simulink model "IEEE33_TR_TEMPORAL_RECOGNIZABILITY_MASTER"  (R2026b)
settings: Solver=ode23t  StopTime=0.2  MaxStep=1e-5
undefined symbols (not defined in the file): Three_PhaseBreaker_class, Three_PhaseSeriesRLCLoad_class, Three_PhaseSource_class, Three_PhaseV_IMeasuremen_class
libraries: ee_lib x146, nesl_utility x106, fl_lib x33, eeRmsMeasurement x2
(part 1 of 7)
settings Model: Creator=JY Wong  LastModifiedBy=sola
settings DataIOCC: ReturnWorkspaceOutputs=off
settings DebuggingCC: ArithmeticOperatorsInVariantConditions=warning  PregeneratedLibrarySubsystemCodeDiagnostic=none  SaveWithParameterizedLinksMsg=none
settings SFSimCC: CustomCodeUndefinedFunction=UseInterfaceOnly  SimUseLocalCustomCode=off
settings RTWCC: RTWUseLocalCustomCode=off
settings SimscapeCC: SimscapeNominalValues="[{\"value\":\"1\",\"unit\":\"A\"},{\"value\":\"1\",\"unit\":\"bar\"},{\"value\":\"1\",\"unit\":\"cm^2\"},{\"value\":\"1\",\"unit\":\"cm^3/s\"},{\"value\":\"1\",\"unit\":\"kJ/kg\"},{\"value\":\"1\",\"unit\":\"kW\"},{\"value\":\"1\",\"unit\":\"l\"},{\"value\":\"1\",\"unit\":\"N\"},{\"value\":\"1\",\"unit\":\"N*m\"},{\"value\":\"1\",\"unit\":\"V\"},{\"value\":\"0.001\",\"unit\":\"Wb\"}]"  SimscapeUseEnergyAccounting=off

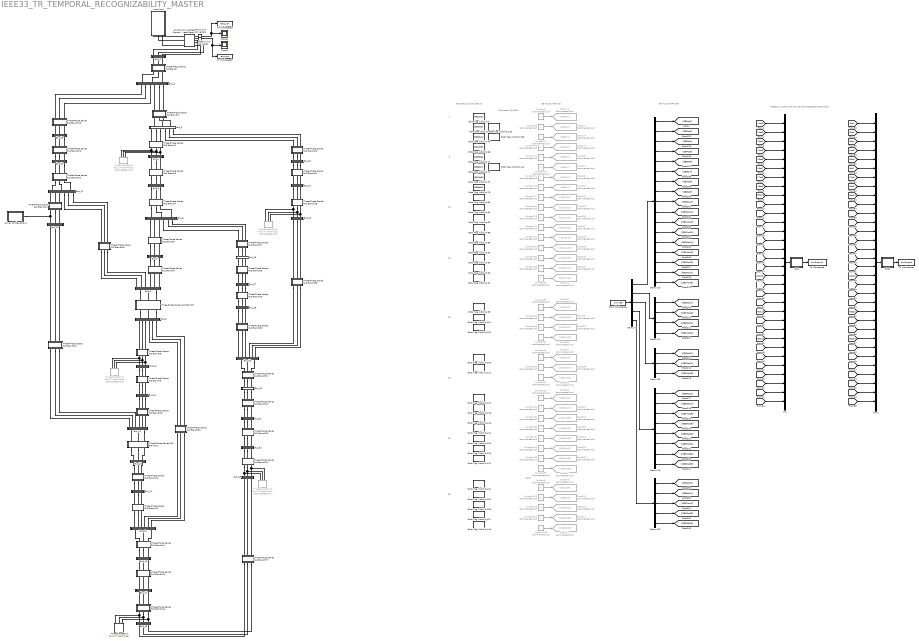
== system IEEE33_TR_TEMPORAL_RECOGNIZABILITY_MASTER ==
  note: NoPs
  note: 33 buses + 5 NOPs
  note: Goto Tag Visibility Blocks
  note: 1
  note: 5
  note: 10
  note: 15
  note: 20
  note: 25
  note: 30
  note: CB Inputs (Manual)
  note: CB Inputs (MATLAB)
  note: Voltage & Current Monitoring at the Respective Branches
  note: 35
  Bus_1 : Subsystem
  Bus_10 : Subsystem
  Bus_11 : Subsystem
  Bus_12 : Subsystem
  Bus_13 : Subsystem
  Bus_14 : Subsystem
  Bus_15 : Subsystem
  Bus_16 : Subsystem
  Bus_17 : Subsystem
  Bus_18 : Subsystem
  Bus_19 : Subsystem
  Bus_2 : Subsystem
  Bus_20 : Subsystem
  Bus_21 : Subsystem
  Bus_22 : Subsystem
  Bus_23 : Subsystem
  Bus_24 : Subsystem
  Bus_25 : Subsystem
  Bus_26 : Subsystem
  Bus_27 : Subsystem
  Bus_28 : Subsystem
  Bus_29 : Subsystem
  Bus_3 : Subsystem
  Bus_30 : Subsystem
  Bus_31 : Subsystem
  Bus_32 : Subsystem
  Bus_33 : Subsystem
  Bus_4 : Subsystem
  Bus_5 : Subsystem
  Bus_6 : Subsystem
  Bus_7 : Subsystem
  Bus_8 : Subsystem
  Bus_9 : Subsystem
  Constant{7..8,71..100} (32 alike) : Constant  Commented=on
  Constant{3..4,133..135} (5 alike) : Constant  Commented=on  Value=0
  Current and Voltage Sensor (Three-Phase) : ee_lib/Sensors & Transducers/Current and Voltage Sensor (Three-Phase)  port_option=ee.enum.threePhasePort.expanded  vMeasurementType=ee.enum.vmeasurement.lg  outputUnit=ee.enum.unit.si  SRated=100e6 A*V  VRated=24e3 V  I_specify=off  I_priority=None  I=[0, 0, 0] A  I_nominal_specify=off  I_nominal_value=1  I_nominal_unit=A  V_specify=off  V_priority=None  V=[0, 0, 0] V  V_nominal_specify=off  V_nominal_value=1  V_nominal_unit=V
  Demux1 : Demux  Outputs=[17,4,3,8,5]
  Demux13 : Demux  Outputs=17
  Demux14 : Demux
  Demux15 : Demux  Outputs=3
  Demux16 : Demux  Outputs=8
  Demux20 : Demux  Outputs=5
  From Workspace1 : FromWorkspace  VariableName=siminCB
  Goto Tag Visibility : GotoTagVisibility  GotoTag=CB2to3
  Goto Tag Visibility102 : GotoTagVisibility  GotoTag=CB21to22
  Goto Tag Visibility104 : GotoTagVisibility  GotoTag=CB20to21
  Goto Tag Visibility106 : GotoTagVisibility  GotoTag=CB23to24
  Goto Tag Visibility110 : GotoTagVisibility  GotoTag=CB26to27
  Goto Tag Visibility112 : GotoTagVisibility  GotoTag=CB24to25
  Goto Tag Visibility114 : GotoTagVisibility  GotoTag=CB6to26
  Goto Tag Visibility116 : GotoTagVisibility  GotoTag=CB28to29
  Goto Tag Visibility118 : GotoTagVisibility  GotoTag=CB27to28
  Goto Tag Visibility120 : GotoTagVisibility  GotoTag=CB30to31
  Goto Tag Visibility122 : GotoTagVisibility  GotoTag=CB29to30
  Goto Tag Visibility124 : GotoTagVisibility  GotoTag=CB32to33
  Goto Tag Visibility126 : GotoTagVisibility  GotoTag=CB31to32
  Goto Tag Visibility129 : GotoTagVisibility  GotoTag=CB2to19
  Goto Tag Visibility130 : GotoTagVisibility  GotoTag=CB3to23
  Goto Tag Visibility132 : GotoTagVisibility  GotoTag=CB9to15
  Goto Tag Visibility134 : GotoTagVisibility  GotoTag=CB21to8
  Goto Tag Visibility136 : GotoTagVisibility  GotoTag=CB22to12
  Goto Tag Visibility137 : GotoTagVisibility  GotoTag=CB18to33
  Goto Tag Visibility140 : GotoTagVisibility  GotoTag=CB25to29
  Goto Tag Visibility4 : GotoTagVisibility  GotoTag=CB1to2
  Goto Tag Visibility68 : GotoTagVisibility  GotoTag=CB4to5
  Goto Tag Visibility70 : GotoTagVisibility  GotoTag=CB3to4
  Goto Tag Visibility72 : GotoTagVisibility  GotoTag=CB6to7
  Goto Tag Visibility74 : GotoTagVisibility  GotoTag=CB5to6
  Goto Tag Visibility76 : GotoTagVisibility  GotoTag=CB8to9
  Goto Tag Visibility78 : GotoTagVisibility  GotoTag=CB7to8
  Goto Tag Visibility80 : GotoTagVisibility  GotoTag=CB9to10
  Goto Tag Visibility82 : GotoTagVisibility  GotoTag=CB11to12
  Goto Tag Visibility84 : GotoTagVisibility  GotoTag=CB10to11
  Goto Tag Visibility86 : GotoTagVisibility  GotoTag=CB13to14
  Goto Tag Visibility88 : GotoTagVisibility  GotoTag=CB12to13
  Goto Tag Visibility90 : GotoTagVisibility  GotoTag=CB15to16
  Goto Tag Visibility92 : GotoTagVisibility  GotoTag=CB14to15
  Goto Tag Visibility94 : GotoTagVisibility  GotoTag=CB17to18
  Goto Tag Visibility96 : GotoTagVisibility  GotoTag=CB16to17
  Goto Tag Visibility98 : GotoTagVisibility  GotoTag=CB19to20
  Goto276 : Goto  Commented=on  GotoTag=CB1to2  TagVisibility=scoped
  Goto277 : Goto  Commented=on  GotoTag=CB2to3  TagVisibility=scoped
  Goto278 : Goto  Commented=on  GotoTag=CB3to4  TagVisibility=scoped
  Goto279 : Goto  Commented=on  GotoTag=CB4to5  TagVisibility=scoped
  Goto280 : Goto  Commented=on  GotoTag=CB5to6  TagVisibility=scoped
  Goto281 : Goto  Commented=on  GotoTag=CB6to7  TagVisibility=scoped
  Goto282 : Goto  Commented=on  GotoTag=CB7to8  TagVisibility=scoped
  Goto283 : Goto  Commented=on  GotoTag=CB8to9  TagVisibility=scoped
  Goto284 : Goto  Commented=on  GotoTag=CB9to10  TagVisibility=scoped
  Goto285 : Goto  Commented=on  GotoTag=CB10to11  TagVisibility=scoped
  Goto286 : Goto  Commented=on  GotoTag=CB11to12  TagVisibility=scoped
  Goto287 : Goto  Commented=on  GotoTag=CB12to13  TagVisibility=scoped
  Goto288 : Goto  Commented=on  GotoTag=CB13to14  TagVisibility=scoped
  Goto289 : Goto  Commented=on  GotoTag=CB14to15  TagVisibility=scoped
  Goto290 : Goto  Commented=on  GotoTag=CB15to16  TagVisibility=scoped
  Goto291 : Goto  Commented=on  GotoTag=CB16to17  TagVisibility=scoped
  Goto292 : Goto  Commented=on  GotoTag=CB2to19  TagVisibility=scoped
  Goto293 : Goto  Commented=on  GotoTag=CB19to20  TagVisibility=scoped
  Goto294 : Goto  Commented=on  GotoTag=CB20to21  TagVisibility=scoped
  Goto295 : Goto  Commented=on  GotoTag=CB21to22  TagVisibility=scoped
  Goto296 : Goto  Commented=on  GotoTag=CB17to18  TagVisibility=scoped
  Goto297 : Goto  Commented=on  GotoTag=CB3to23  TagVisibility=scoped
  Goto298 : Goto  Commented=on  GotoTag=CB23to24  TagVisibility=scoped
  Goto299 : Goto  Commented=on  GotoTag=CB24to25  TagVisibility=scoped
  Goto300 : Goto  Commented=on  GotoTag=CB6to26  TagVisibility=scoped
  Goto301 : Goto  Commented=on  GotoTag=CB26to27  TagVisibility=scoped
  Goto302 : Goto  Commented=on  GotoTag=CB27to28  TagVisibility=scoped
  Goto303 : Goto  Commented=on  GotoTag=CB28to29  TagVisibility=scoped
  Goto304 : Goto  Commented=on  GotoTag=CB29to30  TagVisibility=scoped
  Goto305 : Goto  Commented=on  GotoTag=CB30to31  TagVisibility=scoped
  Goto306 : Goto  Commented=on  GotoTag=CB31to32  TagVisibility=scoped
  Goto307 : Goto  Commented=on  GotoTag=CB32to33  TagVisibility=scoped
  Goto308 : Goto  Commented=on  GotoTag=CB21to8  TagVisibility=scoped
  Goto309 : Goto  Commented=on  GotoTag=CB9to15  TagVisibility=scoped
  Goto310 : Goto  Commented=on  GotoTag=CB22to12  TagVisibility=scoped
  Goto311 : Goto  Commented=on  GotoTag=CB18to33  TagVisibility=scoped
  Goto312 : Goto  Commented=on  GotoTag=CB25to29  TagVisibility=scoped
  Incoming1 : Subsystem
  Mux : Mux  Inputs=32
  Mux1 : Mux  Inputs=32
  PS-Simulink Converter : nesl_utility/PS-Simulink Converter  PhysicalDomain=network_engine_domain  SubClassName=ps_output  LeftPortType=input  RightPortType=output  PseudoPeriodic=off  Frequencies=[]  VectorFormat=inherit  Unit=inherit  AffineConversion=off
  PS-Simulink Converter1 : nesl_utility/PS-Simulink Converter  PhysicalDomain=network_engine_domain  SubClassName=ps_output  LeftPortType=input  RightPortType=output  PseudoPeriodic=off  Frequencies=[]  VectorFormat=inherit  Unit=inherit  AffineConversion=off
  RMS : Subsystem
      settings: OpenFcn=elec.conv.unmask(gcb);
  RMS1 : Subsystem
      settings: OpenFcn=elec.conv.unmask(gcb);
  Scope : Scope
      settings: ActiveDisplayYMinimum=-377.76200799670079  ActiveDisplayYMaximum=376.93956006483484
  Scope1 : Scope
      settings: ActiveDisplayYMinimum=-12921.058393181265  ActiveDisplayYMaximum=12921.058393181265
  Solver Configuration1 : Subsystem  Priority=1
  Three-Phase Series RLC Branch : Subsystem
      settings: AttributesFormatString=\n  OpenFcn=elec.conv.unmask(gcb);
  Three-Phase Series RLC Branch1 : Subsystem
      settings: AttributesFormatString=\n  OpenFcn=elec.conv.unmask(gcb);
  Three-Phase Series RLC Branch10 : Subsystem
      settings: AttributesFormatString=\n  OpenFcn=elec.conv.unmask(gcb);
  Three-Phase Series RLC Branch11 : Subsystem
      settings: AttributesFormatString=\n  OpenFcn=elec.conv.unmask(gcb);
  Three-Phase Series RLC Branch12 : Subsystem
      settings: AttributesFormatString=\n  OpenFcn=elec.conv.unmask(gcb);
  Three-Phase Series RLC Branch13 : Subsystem
      settings: AttributesFormatString=\n  OpenFcn=elec.conv.unmask(gcb);
  Three-Phase Series RLC Branch14 : Subsystem
      settings: AttributesFormatString=\n  OpenFcn=elec.conv.unmask(gcb);
  Three-Phase Series RLC Branch15 : Subsystem
      settings: AttributesFormatString=\n  OpenFcn=elec.conv.unmask(gcb);
  Three-Phase Series RLC Branch16 : Subsystem
      settings: AttributesFormatString=\n  OpenFcn=elec.conv.unmask(gcb);
  Three-Phase Series RLC Branch18 : Subsystem
      settings: AttributesFormatString=\n  OpenFcn=elec.conv.unmask(gcb);
  Three-Phase Series RLC Branch19 : Subsystem
      settings: AttributesFormatString=\n  OpenFcn=elec.conv.unmask(gcb);
  Three-Phase Series RLC Branch2 : Subsystem
      settings: AttributesFormatString=\n  OpenFcn=elec.conv.unmask(gcb);
  Three-Phase Series RLC Branch20 : Subsystem
      settings: AttributesFormatString=\n  OpenFcn=elec.conv.unmask(gcb);
  Three-Phase Series RLC Branch21 : Subsystem
      settings: AttributesFormatString=\n  OpenFcn=elec.conv.unmask(gcb);
  Three-Phase Series RLC Branch22 : Subsystem
      settings: AttributesFormatString=\n  OpenFcn=elec.conv.unmask(gcb);
  Three-Phase Series RLC Branch23 : Subsystem
      settings: AttributesFormatString=\n  OpenFcn=elec.conv.unmask(gcb);
  Three-Phase Series RLC Branch24 : Subsystem
      settings: AttributesFormatString=\n  OpenFcn=elec.conv.unmask(gcb);
  Three-Phase Series RLC Branch25 : Subsystem
      settings: AttributesFormatString=\n  OpenFcn=elec.conv.unmask(gcb);
  Three-Phase Series RLC Branch27 : Subsystem
      settings: AttributesFormatString=\n  OpenFcn=elec.conv.unmask(gcb);
  Three-Phase Series RLC Branch28 : Subsystem
      settings: AttributesFormatString=\n  OpenFcn=elec.conv.unmask(gcb);
  Three-Phase Series RLC Branch29 : Subsystem
      settings: AttributesFormatString=\n  OpenFcn=elec.conv.unmask(gcb);
  Three-Phase Series RLC Branch3 : Subsystem
      settings: AttributesFormatString=\n  OpenFcn=elec.conv.unmask(gcb);
  Three-Phase Series RLC Branch30 : Subsystem
      settings: AttributesFormatString=\n  OpenFcn=elec.conv.unmask(gcb);
  Three-Phase Series RLC Branch31 : Subsystem
      settings: AttributesFormatString=\n  OpenFcn=elec.conv.unmask(gcb);
  Three-Phase Series RLC Branch32 : Subsystem
      settings: AttributesFormatString=\n  OpenFcn=elec.conv.unmask(gcb);
  Three-Phase Series RLC Branch33 : Subsystem
      settings: AttributesFormatString=\n  OpenFcn=elec.conv.unmask(gcb);
  Three-Phase Series RLC Branch34 : Subsystem
      settings: AttributesFormatString=\n  OpenFcn=elec.conv.unmask(gcb);
  Three-Phase Series RLC Branch35 : Subsystem
      settings: AttributesFormatString=\n  OpenFcn=elec.conv.unmask(gcb);
  Three-Phase Series RLC Branch36 : Subsystem
      settings: AttributesFormatString=\n  OpenFcn=elec.conv.unmask(gcb);
  Three-Phase Series RLC Branch37 : Subsystem
      settings: AttributesFormatString=\n  OpenFcn=elec.conv.unmask(gcb);
  Three-Phase Series RLC Branch38 : Subsystem
      settings: AttributesFormatString=\n  OpenFcn=elec.conv.unmask(gcb);
  Three-Phase Series RLC Branch4 : Subsystem
      settings: AttributesFormatString=\n  OpenFcn=elec.conv.unmask(gcb);
  Three-Phase Series RLC Branch5 : Subsystem
      settings: AttributesFormatString=\n  OpenFcn=elec.conv.unmask(gcb);
  Three-Phase Series RLC Branch6 : Subsystem
      settings: AttributesFormatString=\n  OpenFcn=elec.conv.unmask(gcb);
  Three-Phase Series RLC Branch7 : Subsystem
      settings: AttributesFormatString=\n  OpenFcn=elec.conv.unmask(gcb);
  Three-Phase Series RLC Branch8 : Subsystem
      settings: AttributesFormatString=\n  OpenFcn=elec.conv.unmask(gcb);
  Three-Phase Series RLC Branch9 : Subsystem
      settings: AttributesFormatString=\n  OpenFcn=elec.conv.unmask(gcb);
  ThreePhaseFault : ee_lib/Utilities/Fault (Three-Phase)  port_option=ee.enum.threePhasePort.expanded  fault_type_option=ee.enum.fault_type_option.none  R_pn_fault=0.999 Ohm  R_ng_fault=0.001 Ohm  exposemeasurement=ee.enum.exposemeasurement.hidden  enable_external_fault=ee.enum.external_fault.hidden  fault_threshold=0.5  fault_condition=ee.enum.fault_condition.fgt  fault_resettable=ee.enum.enable.no  enable_temporal_fault=ee.enum.enable.yes  fault_start_time=0.1 s  fault_duration=inf s  G_parasitic=1e-4 1/Ohm  I_specify=off  I_priority=None  I=[0, 0, 0] A  I_nominal_specify=off  I_nominal_value=1  I_nominal_unit=A  i_ng_specify=off  i_ng_priority=None  i_ng=0 A  i_ng_nominal_specify=off  i_ng_nominal_value=1  i_ng_nominal_unit=A
  ThreePhaseFault{1..4} (4 alike) : ee_lib/Utilities/Fault (Three-Phase)  Commented=on  port_option=ee.enum.threePhasePort.expanded  fault_type_option=ee.enum.fault_type_option.none  R_pn_fault=0.999 Ohm  R_ng_fault=0.001 Ohm  exposemeasurement=ee.enum.exposemeasurement.hidden  enable_external_fault=ee.enum.external_fault.hidden  fault_threshold=0.5  fault_condition=ee.enum.fault_condition.fgt  fault_resettable=ee.enum.enable.no  enable_temporal_fault=ee.enum.enable.yes  fault_start_time=0.1 s  fault_duration=inf s  G_parasitic=1e-4 1/Ohm  I_specify=off  I_priority=None  I=[0, 0, 0] A  I_nominal_specify=off  I_nominal_value=1  I_nominal_unit=A  i_ng_specify=off  i_ng_priority=None  i_ng=0 A  i_ng_nominal_specify=off  i_ng_nominal_value=1  i_ng_nominal_unit=A
  To Workspace : ToWorkspace  VariableName=simOutputV  SaveFormat=Timeseries  SampleTime=-1
  To Workspace1 : ToWorkspace  VariableName=simOutputI  SaveFormat=Timeseries  SampleTime=-1
  To Workspace2 : ToWorkspace  VariableName=Iabc_raw  SaveFormat=Timeseries  SampleTime=-1
  To Workspace3 : ToWorkspace  VariableName=Vabc_raw  SaveFormat=Timeseries  SampleTime=-1
  tag scope: CB10to11=scoped, CB11to12=scoped, CB12to13=scoped, CB13to14=scoped, CB14to15=scoped, CB15to16=scoped, CB16to17=scoped, CB17to18=scoped, CB18to33=scoped, CB19to20=scoped, CB1to2=scoped, CB20to21=scoped, CB21to22=scoped, CB21to8=scoped, CB22to12=scoped, CB23to24=scoped, CB24to25=scoped, CB25to29=scoped, CB26to27=scoped, CB27to28=scoped, CB28to29=scoped, CB29to30=scoped, CB2to19=scoped, CB2to3=scoped, CB30to31=scoped, CB31to32=scoped, CB32to33=scoped, CB3to23=scoped, CB3to4=scoped, CB4to5=scoped, CB5to6=scoped, CB6to26=scoped, CB6to7=scoped, CB7to8=scoped, CB8to9=scoped, CB9to10=scoped, CB9to15=scoped
  wires:
  Constant7/1 -> Goto276/1
  Constant8/1 -> Goto277/1
  Constant71/1 -> Goto278/1
  Constant72/1 -> Goto279/1
  Constant73/1 -> Goto280/1
  Constant76/1 -> Goto281/1
  Constant75/1 -> Goto283/1
  Constant74/1 -> Goto282/1
  Constant77/1 -> Goto284/1
  Constant80/1 -> Goto285/1
  Constant79/1 -> Goto287/1
  Constant78/1 -> Goto286/1
  Constant81/1 -> Goto288/1
  Constant84/1 -> Goto289/1
  Constant83/1 -> Goto291/1
  Constant82/1 -> Goto290/1
  Constant85/1 -> Goto292/1
  Constant88/1 -> Goto293/1
  Constant87/1 -> Goto295/1
  Constant86/1 -> Goto294/1
  Constant91/1 -> Goto299/1
  Constant93/1 -> Goto298/1
  Constant90/1 -> Goto297/1
  Constant94/1 -> Goto302/1
  Constant95/1 -> Goto303/1
  Constant96/1 -> Goto301/1
  Constant92/1 -> Goto300/1
  Constant98/1 -> Goto306/1
  Constant99/1 -> Goto307/1
  Constant100/1 -> Goto305/1
  Constant97/1 -> Goto304/1
  Constant89/1 -> Goto296/1
  From Workspace1/1 -> Demux1/1
  Demux14/2 -> [CB19to20]
  Demux13/17 -> [CB17to18]
  Demux16/5 -> [CB29to30]
  Demux16/8 -> [CB32to33]
  Demux13/15 -> [CB15to16]
  Demux13/5 -> [CB5to6]
  Demux13/11 -> [CB11to12]
  Demux13/10 -> [CB10to11]
  Demux16/7 -> [CB31to32]
  Demux15/2 -> [CB23to24]
  Demux13/3 -> [CB3to4]
  Demux13/4 -> [CB4to5]
  Demux13/16 -> [CB16to17]
  Demux13/6 -> [CB6to7]
  Demux13/1 -> [CB1to2]
  Demux15/3 -> [CB24to25]
  Demux16/2 -> [CB26to27]
  Demux1/4 -> Demux16/1
  Demux13/13 -> [CB13to14]
  Demux14/1 -> [CB2to19]
  Demux13/8 -> [CB8to9]
  Demux1/1 -> Demux13/1
  Demux16/3 -> [CB27to28]
  Demux13/12 -> [CB12to13]
  Demux13/14 -> [CB14to15]
  Demux16/6 -> [CB30to31]
  Demux13/2 -> [CB2to3]
  Demux13/7 -> [CB7to8]
  Demux1/3 -> Demux15/1
  Demux14/3 -> [CB20to21]
  Demux16/1 -> [CB6to26]
  Demux1/2 -> Demux14/1
  Demux13/9 -> [CB9to10]
  Demux16/4 -> [CB28to29]
  Demux14/4 -> [CB21to22]
  Demux15/1 -> [CB3to23]
  Mux/1 -> RMS/1(In)
  RMS/1(RMS) -> To Workspace/1
  RMS1/1(RMS) -> To Workspace1/1
  Mux1/1 -> RMS1/1(In)
  [I4to5] -> Mux1/4
  [I24to25] -> Mux1/24
  [I6to26] -> Mux1/25
  [I26to27] -> Mux1/26
  [I5to6] -> Mux1/5
  [I7to8] -> Mux1/7
  [I6to7] -> Mux1/6
  [I8to9] -> Mux1/8
  [I9to10] -> Mux1/9
  [I10to11] -> Mux1/10
  [I17to18] -> Mux1/17
  [I2to19] -> Mux1/18
  [I27to28] -> Mux1/27
  [I28to29] -> Mux1/28
  [I3to4] -> Mux1/3
  [I29to30] -> Mux1/29
  [I31to32] -> Mux1/31
  [I30to31] -> Mux1/30
  [I32to33] -> Mux1/32
  [I19to20] -> Mux1/19
  [I20to21] -> Mux1/20
  [I3to23] -> Mux1/22
  [I21to22] -> Mux1/21
  [I23to24] -> Mux1/23
  [I15to16] -> Mux1/15
  [I14to15] -> Mux1/14
  [I16to17] -> Mux1/16
  [I2to3] -> Mux1/2
  [I13to14] -> Mux1/13
  [I12to13] -> Mux1/12
  [I11to12] -> Mux1/11
  [V32to33] -> Mux/32
  Demux20/5 -> [CB25to29]
  Demux20/3 -> [CB22to12]
  Demux20/2 -> [CB9to15]
  Demux20/4 -> [CB18to33]
  Demux20/1 -> [CB21to8]
  Demux1/5 -> Demux20/1
  Constant4/1 -> Goto308/1
  Constant133/1 -> Goto309/1
  Constant3/1 -> Goto310/1
  Constant134/1 -> Goto311/1
  Constant135/1 -> Goto312/1
  [V31to32] -> Mux/31
  [V30to31] -> Mux/30
  [V29to30] -> Mux/29
  [V28to29] -> Mux/28
  [V27to28] -> Mux/27
  [V26to27] -> Mux/26
  [V6to26] -> Mux/25
  [V24to25] -> Mux/24
  [V23to24] -> Mux/23
  [V3to23] -> Mux/22
  [V21to22] -> Mux/21
  [V20to21] -> Mux/20
  [V19to20] -> Mux/19
  [V2to19] -> Mux/18
  [V17to18] -> Mux/17
  [V16to17] -> Mux/16
  [V15to16] -> Mux/15
  [V14to15] -> Mux/14
  [V13to14] -> Mux/13
  [V12to13] -> Mux/12
  [V11to12] -> Mux/11
  [V10to11] -> Mux/10
  [V9to10] -> Mux/9
  [V8to9] -> Mux/8
  [V6to7] -> Mux/6
  [V7to8] -> Mux/7
  [V5to6] -> Mux/5
  [V4to5] -> Mux/4
  [V3to4] -> Mux/3
  [V2to3] -> Mux/2
  [V1to2] -> Mux/1
  [I1to2] -> Mux1/1
  PS-Simulink Converter1/1 -> To Workspace3/1, Scope1/1
  PS-Simulink Converter/1 -> To Workspace2/1, Scope/1
  connections:
  Bus_1/RConn2 -- Three-Phase Series RLC Branch/LConn2
  Bus_3/RConn2 -- Three-Phase Series RLC Branch2/LConn2
  Bus_3/RConn3 -- Three-Phase Series RLC Branch2/LConn3
  Bus_3/RConn1 -- Three-Phase Series RLC Branch2/LConn1
  Bus_4/RConn2 -- Three-Phase Series RLC Branch3/LConn2
  Bus_5/RConn2 -- Three-Phase Series RLC Branch4/LConn2
  Bus_5/RConn3 -- Three-Phase Series RLC Branch4/LConn3
  Bus_5/RConn1 -- Three-Phase Series RLC Branch4/LConn1
  Three-Phase Series RLC Branch5/LConn3 -- Bus_6/RConn3
  Bus_7/RConn3 -- Three-Phase Series RLC Branch6/LConn3
  Bus_9/RConn1 -- Three-Phase Series RLC Branch8/LConn1
  Bus_19/RConn3 -- Three-Phase Series RLC Branch19/LConn3
  Bus_20/RConn3 -- Three-Phase Series RLC Branch20/LConn3
  Bus_23/RConn3 -- Three-Phase Series RLC Branch24/LConn3
  Bus_27/RConn3 -- Three-Phase Series RLC Branch29/LConn3
  Bus_27/RConn2 -- Three-Phase Series RLC Branch29/LConn2
  Three-Phase Series RLC Branch35/RConn1 -- Bus_8/LConn1
  Three-Phase Series RLC Branch35/RConn2 -- Bus_8/LConn2
  Three-Phase Series RLC Branch35/RConn3 -- Bus_8/LConn3
  Bus_3/LConn1 -- Three-Phase Series RLC Branch1/RConn1
  Bus_3/LConn2 -- Three-Phase Series RLC Branch1/RConn2
  Bus_3/LConn3 -- Three-Phase Series RLC Branch1/RConn3
  Bus_19/LConn3 -- Three-Phase Series RLC Branch18/RConn3
  Bus_19/LConn2 -- Three-Phase Series RLC Branch18/RConn2
  Bus_19/LConn1 -- Three-Phase Series RLC Branch18/RConn1
  Three-Phase Series RLC Branch19/LConn1 -- Bus_19/RConn1
  Three-Phase Series RLC Branch19/LConn2 -- Bus_19/RConn2
  Bus_20/RConn2 -- Three-Phase Series RLC Branch20/LConn2
  Bus_20/LConn3 -- Three-Phase Series RLC Branch19/RConn3
  Three-Phase Series RLC Branch19/RConn2 -- Bus_20/LConn2
  Three-Phase Series RLC Branch19/RConn1 -- Bus_20/LConn1
  Three-Phase Series RLC Branch20/LConn1 -- Bus_20/RConn1
  Three-Phase Series RLC Branch20/RConn3 -- Bus_21/LConn3
  Three-Phase Series RLC Branch20/RConn2 -- Bus_21/LConn2
  Three-Phase Series RLC Branch20/RConn1 -- Bus_21/LConn1
  Three-Phase Series RLC Branch21/LConn1 -- Bus_21/RConn1
  Three-Phase Series RLC Branch21/LConn2 -- Bus_21/RConn2
  Three-Phase Series RLC Branch21/LConn3 -- Bus_21/RConn3
  Bus_22/LConn3 -- Three-Phase Series RLC Branch21/RConn3
  Three-Phase Series RLC Branch21/RConn1 -- Bus_22/LConn1 -- Solver Configuration1/RConn1
  Bus_22/RConn1 -- Three-Phase Series RLC Branch22/LConn1
  Bus_22/RConn2 -- Three-Phase Series RLC Branch22/LConn2
  Bus_22/RConn3 -- Three-Phase Series RLC Branch22/LConn3
  Three-Phase Series RLC Branch3/LConn3 -- Bus_4/RConn3
  Bus_4/LConn3 -- ThreePhaseFault2/LConn3 -- Three-Phase Series RLC Branch2/RConn3
  Three-Phase Series RLC Branch2/RConn2 -- ThreePhaseFault2/LConn2 -- Bus_4/LConn2
  Three-Phase Series RLC Branch2/RConn1 -- ThreePhaseFault2/LConn1 -- Bus_4/LConn1
  Three-Phase Series RLC Branch3/LConn1 -- Bus_4/RConn1
  Bus_2/LConn3 -- Three-Phase Series RLC Branch/RConn3
  Three-Phase Series RLC Branch/RConn2 -- Bus_2/LConn2
  Bus_2/LConn1 -- Three-Phase Series RLC Branch/RConn1
  Bus_5/LConn3 -- Three-Phase Series RLC Branch3/RConn3
  Three-Phase Series RLC Branch3/RConn2 -- Bus_5/LConn2
  Three-Phase Series RLC Branch3/RConn1 -- Bus_5/LConn1
  Bus_6/LConn3 -- Three-Phase Series RLC Branch4/RConn3
  Three-Phase Series RLC Branch4/RConn2 -- Bus_6/LConn2
  Three-Phase Series RLC Branch4/RConn1 -- Bus_6/LConn1
  Bus_6/RConn1 -- Three-Phase Series RLC Branch5/LConn1
  Three-Phase Series RLC Branch5/LConn2 -- Bus_6/RConn2
  Bus_7/LConn3 -- Three-Phase Series RLC Branch5/RConn3
  Three-Phase Series RLC Branch5/RConn2 -- Bus_7/LConn2
  Three-Phase Series RLC Branch5/RConn1 -- Bus_7/LConn1
  Bus_7/RConn1 -- Three-Phase Series RLC Branch6/LConn1
  Bus_7/RConn2 -- Three-Phase Series RLC Branch6/LConn2
  Three-Phase Series RLC Branch7/RConn3 -- Bus_9/LConn3
  Bus_9/LConn2 -- Three-Phase Series RLC Branch7/RConn2
  Three-Phase Series RLC Branch7/RConn1 -- Bus_9/LConn1
  Bus_9/RConn2 -- Three-Phase Series RLC Branch8/LConn2
  Bus_9/RConn3 -- Three-Phase Series RLC Branch8/LConn3
  Bus_10/LConn3 -- ThreePhaseFault1/LConn3 -- Three-Phase Series RLC Branch8/RConn3
  Three-Phase Series RLC Branch8/RConn2 -- ThreePhaseFault1/LConn2 -- Bus_10/LConn2
  Three-Phase Series RLC Branch8/RConn1 -- ThreePhaseFault1/LConn1 -- Bus_10/LConn1
  Bus_10/RConn1 -- Three-Phase Series RLC Branch9/LConn1
  Bus_10/RConn2 -- Three-Phase Series RLC Branch9/LConn2
  Three-Phase Series RLC Branch9/LConn3 -- Bus_10/RConn3
  Bus_11/LConn3 -- Three-Phase Series RLC Branch9/RConn3
  Bus_11/RConn3 -- Three-Phase Series RLC Branch10/LConn3
  Three-Phase Series RLC Branch10/LConn2 -- Bus_11/RConn2
  Bus_11/RConn1 -- Three-Phase Series RLC Branch10/LConn1
  Three-Phase Series RLC Branch9/RConn1 -- Bus_11/LConn1
  Three-Phase Series RLC Branch9/RConn2 -- Bus_11/LConn2
  Bus_13/LConn3 -- Three-Phase Series RLC Branch11/RConn3
  Bus_13/RConn3 -- Three-Phase Series RLC Branch12/LConn3
  Bus_13/RConn2 -- Three-Phase Series RLC Branch12/LConn2
  Three-Phase Series RLC Branch11/RConn2 -- Bus_13/LConn2
  Three-Phase Series RLC Branch11/RConn1 -- Bus_13/LConn1
  Bus_13/RConn1 -- Three-Phase Series RLC Branch12/LConn1
  Bus_14/LConn3 -- Three-Phase Series RLC Branch12/RConn3
  Three-Phase Series RLC Branch13/LConn3 -- Bus_14/RConn3
  Three-Phase Series RLC Branch12/RConn2 -- Bus_14/LConn2
  Three-Phase Series RLC Branch12/RConn1 -- Bus_14/LConn1
  Three-Phase Series RLC Branch13/LConn1 -- Bus_14/RConn1
  Bus_14/RConn2 -- Three-Phase Series RLC Branch13/LConn2
  Bus_15/LConn3 -- Three-Phase Series RLC Branch13/RConn3
  Three-Phase Series RLC Branch13/RConn2 -- Bus_15/LConn2
  Three-Phase Series RLC Branch13/RConn1 -- Bus_15/LConn1
  Bus_16/LConn3 -- Three-Phase Series RLC Branch14/RConn3
  Three-Phase Series RLC Branch14/RConn2 -- Bus_16/LConn2
  Three-Phase Series RLC Branch14/RConn1 -- Bus_16/LConn1
  Bus_17/LConn3 -- Three-Phase Series RLC Branch15/RConn3
  Bus_17/LConn2 -- Three-Phase Series RLC Branch15/RConn2
  Bus_17/LConn1 -- Three-Phase Series RLC Branch15/RConn1
  Three-Phase Series RLC Branch16/RConn1 -- Bus_18/LConn1 -- ThreePhaseFault/LConn1
  Bus_23/LConn3 -- Three-Phase Series RLC Branch23/RConn3
  Three-Phase Series RLC Branch23/RConn2 -- Bus_23/LConn2
  Three-Phase Series RLC Branch23/RConn1 -- Bus_23/LConn1
  Bus_23/RConn1 -- Three-Phase Series RLC Branch24/LConn1
  Bus_23/RConn2 -- Three-Phase Series RLC Branch24/LConn2
  Bus_24/LConn3 -- Three-Phase Series RLC Branch24/RConn3
  Bus_24/RConn3 -- Three-Phase Series RLC Branch25/LConn3
  Three-Phase Series RLC Branch24/RConn2 -- Bus_24/LConn2
  Three-Phase Series RLC Branch24/RConn1 -- Bus_24/LConn1
  Bus_24/RConn1 -- Three-Phase Series RLC Branch25/LConn1
  Bus_24/RConn2 -- Three-Phase Series RLC Branch25/LConn2
  Bus_25/LConn3 -- ThreePhaseFault3/LConn3 -- Three-Phase Series RLC Branch25/RConn3
  Three-Phase Series RLC Branch38/LConn3 -- Bus_25/RConn3
  Bus_25/RConn2 -- Three-Phase Series RLC Branch38/LConn2
  Bus_25/RConn1 -- Three-Phase Series RLC Branch38/LConn1
  Three-Phase Series RLC Branch25/RConn1 -- ThreePhaseFault3/LConn1 -- Bus_25/LConn1
  Three-Phase Series RLC Branch25/RConn2 -- ThreePhaseFault3/LConn2 -- Bus_25/LConn2
  Bus_26/LConn3 -- Three-Phase Series RLC Branch27/RConn3
  Three-Phase Series RLC Branch28/LConn3 -- Bus_26/RConn3
  Three-Phase Series RLC Branch27/RConn2 -- Bus_26/LConn2
  Three-Phase Series RLC Branch27/RConn1 -- Bus_26/LConn1
  Bus_26/RConn1 -- Three-Phase Series RLC Branch28/LConn1
  Bus_26/RConn2 -- Three-Phase Series RLC Branch28/LConn2
  Bus_27/LConn3 -- Three-Phase Series RLC Branch28/RConn3
  Three-Phase Series RLC Branch29/LConn1 -- Bus_27/RConn1
  Three-Phase Series RLC Branch28/RConn1 -- Bus_27/LConn1
  Three-Phase Series RLC Branch28/RConn2 -- Bus_27/LConn2
  Bus_28/LConn3 -- Three-Phase Series RLC Branch29/RConn3
  Three-Phase Series RLC Branch29/RConn2 -- Bus_28/LConn2
  Three-Phase Series RLC Branch29/RConn1 -- Bus_28/LConn1
  Three-Phase Series RLC Branch30/LConn3 -- Bus_28/RConn3
  Bus_28/RConn2 -- Three-Phase Series RLC Branch30/LConn2
  Bus_28/RConn1 -- Three-Phase Series RLC Branch30/LConn1
  Bus_29/LConn3 -- Three-Phase Series RLC Branch30/RConn3
  Three-Phase Series RLC Branch30/RConn2 -- Bus_29/LConn2
  Three-Phase Series RLC Branch30/RConn1 -- Bus_29/LConn1
  Bus_29/RConn3 -- Three-Phase Series RLC Branch31/LConn3
  Bus_29/RConn2 -- Three-Phase Series RLC Branch31/LConn2
  Bus_29/RConn1 -- Three-Phase Series RLC Branch31/LConn1
  Bus_30/LConn3 -- Three-Phase Series RLC Branch31/RConn3
  Three-Phase Series RLC Branch31/RConn2 -- Bus_30/LConn2
  Three-Phase Series RLC Branch31/RConn1 -- Bus_30/LConn1
  Bus_30/RConn3 -- Three-Phase Series RLC Branch32/LConn3
  Bus_30/RConn2 -- Three-Phase Series RLC Branch32/LConn2
  Bus_30/RConn1 -- Three-Phase Series RLC Branch32/LConn1
  Bus_31/LConn3 -- Three-Phase Series RLC Branch32/RConn3
  Three-Phase Series RLC Branch33/LConn3 -- Bus_31/RConn3
  Three-Phase Series RLC Branch32/RConn2 -- Bus_31/LConn2
  Three-Phase Series RLC Branch32/RConn1 -- Bus_31/LConn1
  Bus_31/RConn2 -- Three-Phase Series RLC Branch33/LConn2
  Bus_31/RConn1 -- Three-Phase Series RLC Branch33/LConn1
  Bus_32/LConn3 -- Three-Phase Series RLC Branch33/RConn3
  Three-Phase Series RLC Branch33/RConn2 -- Bus_32/LConn2
  Three-Phase Series RLC Branch33/RConn1 -- Bus_32/LConn1
  Three-Phase Series RLC Branch34/LConn3 -- Bus_32/RConn3
  Bus_32/RConn2 -- Three-Phase Series RLC Branch34/LConn2
  Bus_32/RConn1 -- Three-Phase Series RLC Branch34/LConn1
  Bus_33/LConn3 -- ThreePhaseFault4/LConn3 -- Three-Phase Series RLC Branch34/RConn3
  Three-Phase Series RLC Branch34/RConn2 -- ThreePhaseFault4/LConn2 -- Bus_33/LConn2
  Three-Phase Series RLC Branch34/RConn1 -- ThreePhaseFault4/LConn1 -- Bus_33/LConn1
  Three-Phase Series RLC Branch16/RConn3 -- Bus_18/LConn3 -- ThreePhaseFault/LConn3
  Three-Phase Series RLC Branch/LConn1 -- Bus_1/RConn1
  Three-Phase Series RLC Branch/LConn3 -- Bus_1/RConn3
  Bus_6/RConn4 -- Three-Phase Series RLC Branch27/LConn1
  Bus_6/RConn5 -- Three-Phase Series RLC Branch27/LConn2
  Bus_6/RConn6 -- Three-Phase Series RLC Branch27/LConn3
  Three-Phase Series RLC Branch1/LConn3 -- Bus_2/RConn6
  Bus_2/RConn5 -- Three-Phase Series RLC Branch1/LConn2
  Three-Phase Series RLC Branch1/LConn1 -- Bus_2/RConn4
  Three-Phase Series RLC Branch18/LConn3 -- Bus_2/RConn3
  Bus_2/RConn2 -- Three-Phase Series RLC Branch18/LConn2
  Three-Phase Series RLC Branch18/LConn1 -- Bus_2/RConn1
  Bus_3/RConn4 -- Three-Phase Series RLC Branch23/LConn1
  Bus_3/RConn5 -- Three-Phase Series RLC Branch23/LConn2
  Bus_3/RConn6 -- Three-Phase Series RLC Branch23/LConn3
  Bus_8/LConn6 -- Three-Phase Series RLC Branch6/RConn3
  Bus_8/LConn4 -- Three-Phase Series RLC Branch6/RConn1
  Bus_8/LConn5 -- Three-Phase Series RLC Branch6/RConn2
  Bus_8/RConn1 -- Three-Phase Series RLC Branch7/LConn1
  Three-Phase Series RLC Branch7/LConn2 -- Bus_8/RConn2
  Bus_8/RConn3 -- Three-Phase Series RLC Branch7/LConn3
  Bus_21/RConn4 -- Three-Phase Series RLC Branch35/LConn1
  Bus_21/RConn5 -- Three-Phase Series RLC Branch35/LConn2
  Bus_21/RConn6 -- Three-Phase Series RLC Branch35/LConn3
  Three-Phase Series RLC Branch21/RConn2 -- Bus_22/LConn2
  Three-Phase Series RLC Branch36/LConn1 -- Bus_9/RConn4
  Bus_9/RConn5 -- Three-Phase Series RLC Branch36/LConn2
  Three-Phase Series RLC Branch36/LConn3 -- Bus_9/RConn6
  Bus_12/LConn6 -- Three-Phase Series RLC Branch10/RConn3
  Bus_12/LConn5 -- Three-Phase Series RLC Branch10/RConn2
  Bus_12/LConn4 -- Three-Phase Series RLC Branch10/RConn1
  Three-Phase Series RLC Branch22/RConn3 -- Bus_12/LConn3
  Three-Phase Series RLC Branch22/RConn2 -- Bus_12/LConn2
  Three-Phase Series RLC Branch22/RConn1 -- Bus_12/LConn1
  Three-Phase Series RLC Branch11/LConn2 -- Bus_12/RConn2
  Three-Phase Series RLC Branch11/LConn1 -- Bus_12/RConn1
  Bus_12/RConn3 -- Three-Phase Series RLC Branch11/LConn3
  Three-Phase Series RLC Branch36/RConn1 -- Bus_15/LConn4
  Bus_15/LConn5 -- Three-Phase Series RLC Branch36/RConn2
  Three-Phase Series RLC Branch36/RConn3 -- Bus_15/LConn6
  Three-Phase Series RLC Branch14/LConn2 -- Bus_15/RConn2
  Bus_15/RConn1 -- Three-Phase Series RLC Branch14/LConn1
  Three-Phase Series RLC Branch14/LConn3 -- Bus_15/RConn3
  Three-Phase Series RLC Branch15/LConn2 -- Bus_16/RConn2
  Bus_16/RConn1 -- Three-Phase Series RLC Branch15/LConn1
  Three-Phase Series RLC Branch15/LConn3 -- Bus_16/RConn3
  Three-Phase Series RLC Branch16/LConn3 -- Bus_17/RConn3
  Three-Phase Series RLC Branch16/LConn2 -- Bus_17/RConn2
  Three-Phase Series RLC Branch16/LConn1 -- Bus_17/RConn1
  Three-Phase Series RLC Branch38/RConn1 -- Bus_29/LConn4
  Bus_29/LConn5 -- Three-Phase Series RLC Branch38/RConn2
  Three-Phase Series RLC Branch38/RConn3 -- Bus_29/LConn6
  Three-Phase Series RLC Branch37/LConn1 -- Bus_33/RConn1
  Three-Phase Series RLC Branch37/LConn2 -- Bus_33/RConn2
  Three-Phase Series RLC Branch37/LConn3 -- Bus_33/RConn3
  Three-Phase Series RLC Branch37/RConn1 -- Bus_18/RConn1
  Three-Phase Series RLC Branch37/RConn2 -- Bus_18/RConn2
  Three-Phase Series RLC Branch37/RConn3 -- Bus_18/RConn3
  Current and Voltage Sensor (Three-Phase)/LConn1 -- Incoming1/RConn1
  Current and Voltage Sensor (Three-Phase)/LConn2 -- Incoming1/RConn2
  Current and Voltage Sensor (Three-Phase)/LConn3 -- Incoming1/RConn3
  Current and Voltage Sensor (Three-Phase)/RConn5 -- Bus_1/LConn3
  Current and Voltage Sensor (Three-Phase)/RConn4 -- Bus_1/LConn2
  Current and Voltage Sensor (Three-Phase)/RConn3 -- Bus_1/LConn1
  PS-Simulink Converter1/LConn1 -- Current and Voltage Sensor (Three-Phase)/RConn1
  PS-Simulink Converter/LConn1 -- Current and Voltage Sensor (Three-Phase)/RConn2
  Three-Phase Series RLC Branch16/RConn2 -- ThreePhaseFault/LConn2 -- Bus_18/LConn2

== system IEEE33_TR_TEMPORAL_RECOGNIZABILITY_MASTER/Bus_1 ==
  Bus_1 : Subsystem
      settings: OpenFcn=elec.conv.unmask(gcb);
  CB1-2 : Subsystem
      settings: OpenFcn=elec.conv.unmask(gcb);
  Terminator : Terminator
  Terminator1 : Terminator
  InPhaseA : PMIOPort  Side=Left
  InPhaseB : PMIOPort  Port=2  Side=Left
  InPhaseC : PMIOPort  Port=3  Side=Left
  OutPhaseA : PMIOPort  Port=4  Side=Right
  OutPhaseB : PMIOPort  Port=5  Side=Right
  OutPhaseC : PMIOPort  Port=6  Side=Right
  wires:
  [CB1to2] -> CB1-2/1(com)
  Bus_1/1(Vabc) -> Terminator/1
  Bus_1/2(Iabc) -> Terminator1/1
  connections:
  CB1-2/LConn1 -- Bus_1/RConn1
  CB1-2/RConn3 -- OutPhaseC/RConn1
  CB1-2/LConn2 -- Bus_1/RConn2
  CB1-2/LConn3 -- Bus_1/RConn3
  CB1-2/RConn1 -- OutPhaseA/RConn1
  CB1-2/RConn2 -- OutPhaseB/RConn1
  InPhaseA/RConn1 -- Bus_1/LConn1
  InPhaseB/RConn1 -- Bus_1/LConn2
  InPhaseC/RConn1 -- Bus_1/LConn3

== system IEEE33_TR_TEMPORAL_RECOGNIZABILITY_MASTER/Bus_10 ==
  Bus Load 10 : Subsystem
      settings: AttributesFormatString=\n  OpenFcn=elec.conv.unmask(gcb);
  Bus_10 : Subsystem
      settings: OpenFcn=elec.conv.unmask(gcb);
  CB3-2 : Subsystem
      settings: OpenFcn=elec.conv.unmask(gcb);
  VI Recorder13 : Subsystem
  InPhaseA : PMIOPort  Side=Left
  InPhaseB : PMIOPort  Port=2  Side=Left
  InPhaseC : PMIOPort  Port=3  Side=Left
  OutPhaseA : PMIOPort  Port=4  Side=Right
  OutPhaseB : PMIOPort  Port=5  Side=Right
  OutPhaseC : PMIOPort  Port=6  Side=Right
  wires:
  [CB10to11] -> CB3-2/1(com)
  Bus_10/2(Iabc) -> VI Recorder13/2(Irec)
  Bus_10/1(Vabc) -> VI Recorder13/1(Vrec)
  connections:
  Bus_10/RConn1 -- CB3-2/LConn1 -- Bus Load 10/LConn1
  CB3-2/RConn3 -- OutPhaseC/RConn1
  Bus Load 10/LConn2 -- CB3-2/LConn2 -- Bus_10/RConn2
  Bus Load 10/LConn3 -- CB3-2/LConn3 -- Bus_10/RConn3
  CB3-2/RConn1 -- OutPhaseA/RConn1
  CB3-2/RConn2 -- OutPhaseB/RConn1
  InPhaseA/RConn1 -- Bus_10/LConn1
  InPhaseB/RConn1 -- Bus_10/LConn2
  InPhaseC/RConn1 -- Bus_10/LConn3

== system IEEE33_TR_TEMPORAL_RECOGNIZABILITY_MASTER/Bus_11 ==
  Bus Load 11 : Subsystem
      settings: AttributesFormatString=\n  OpenFcn=elec.conv.unmask(gcb);
  Bus_11 : Subsystem
      settings: OpenFcn=elec.conv.unmask(gcb);
  CB3-2 : Subsystem
      settings: OpenFcn=elec.conv.unmask(gcb);
  VI Recorder14 : Subsystem
  InPhaseA : PMIOPort  Side=Left
  InPhaseB : PMIOPort  Port=2  Side=Left
  InPhaseC : PMIOPort  Port=3  Side=Left
  OutPhaseA : PMIOPort  Port=4  Side=Right
  OutPhaseB : PMIOPort  Port=5  Side=Right
  OutPhaseC : PMIOPort  Port=6  Side=Right
  wires:
  [CB11to12] -> CB3-2/1(com)
  Bus_11/2(Iabc) -> VI Recorder14/2(Irec)
  Bus_11/1(Vabc) -> VI Recorder14/1(Vrec)
  connections:
  Bus_11/RConn1 -- CB3-2/LConn1 -- Bus Load 11/LConn1
  CB3-2/RConn3 -- OutPhaseC/RConn1
  Bus Load 11/LConn2 -- CB3-2/LConn2 -- Bus_11/RConn2
  Bus_11/RConn3 -- CB3-2/LConn3 -- Bus Load 11/LConn3
  CB3-2/RConn1 -- OutPhaseA/RConn1
  CB3-2/RConn2 -- OutPhaseB/RConn1
  InPhaseA/RConn1 -- Bus_11/LConn1
  InPhaseB/RConn1 -- Bus_11/LConn2
  InPhaseC/RConn1 -- Bus_11/LConn3

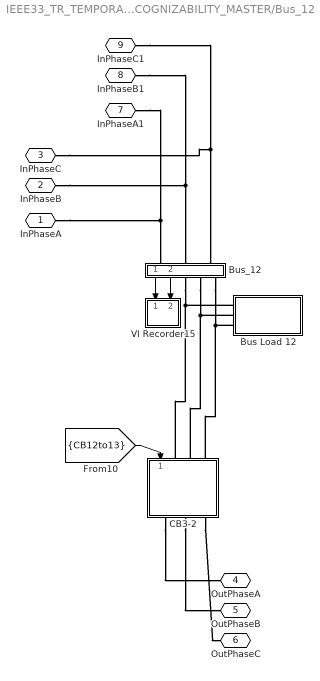
== system IEEE33_TR_TEMPORAL_RECOGNIZABILITY_MASTER/Bus_12 ==
  Bus Load 12 : Subsystem
      settings: AttributesFormatString=\n  OpenFcn=elec.conv.unmask(gcb);
  Bus_12 : Subsystem
      settings: OpenFcn=elec.conv.unmask(gcb);
  CB3-2 : Subsystem
      settings: OpenFcn=elec.conv.unmask(gcb);
  VI Recorder15 : Subsystem
  InPhaseA : PMIOPort  Side=Left
  InPhaseB : PMIOPort  Port=2  Side=Left
  InPhaseC : PMIOPort  Port=3  Side=Left
  OutPhaseA : PMIOPort  Port=4  Side=Right
  OutPhaseB : PMIOPort  Port=5  Side=Right
  OutPhaseC : PMIOPort  Port=6  Side=Right
  InPhaseA1 : PMIOPort  Port=7  Side=Left
  InPhaseB1 : PMIOPort  Port=8  Side=Left
  InPhaseC1 : PMIOPort  Port=9  Side=Left
  wires:
  [CB12to13] -> CB3-2/1(com)
  Bus_12/2(Iabc) -> VI Recorder15/2(Irec)
  Bus_12/1(Vabc) -> VI Recorder15/1(Vrec)
  connections:
  Bus Load 12/LConn1 -- CB3-2/LConn1 -- Bus_12/RConn1
  CB3-2/RConn3 -- OutPhaseC/RConn1
  Bus Load 12/LConn2 -- CB3-2/LConn2 -- Bus_12/RConn2
  Bus Load 12/LConn3 -- CB3-2/LConn3 -- Bus_12/RConn3
  CB3-2/RConn1 -- OutPhaseA/RConn1
  CB3-2/RConn2 -- OutPhaseB/RConn1
  InPhaseA1/RConn1 -- InPhaseA/RConn1 -- Bus_12/LConn1
  InPhaseB1/RConn1 -- InPhaseB/RConn1 -- Bus_12/LConn2
  InPhaseC1/RConn1 -- InPhaseC/RConn1 -- Bus_12/LConn3

== system IEEE33_TR_TEMPORAL_RECOGNIZABILITY_MASTER/Bus_13 ==
  Bus Load 13 : Subsystem
      settings: AttributesFormatString=\n  OpenFcn=elec.conv.unmask(gcb);
  Bus_13 : Subsystem
      settings: OpenFcn=elec.conv.unmask(gcb);
  CB3-2 : Subsystem
      settings: OpenFcn=elec.conv.unmask(gcb);
  VI Recorder16 : Subsystem
  InPhaseA : PMIOPort  Side=Left
  InPhaseB : PMIOPort  Port=2  Side=Left
  InPhaseC : PMIOPort  Port=3  Side=Left
  OutPhaseA : PMIOPort  Port=4  Side=Right
  OutPhaseB : PMIOPort  Port=5  Side=Right
  OutPhaseC : PMIOPort  Port=6  Side=Right
  wires:
  [CB13to14] -> CB3-2/1(com)
  Bus_13/2(Iabc) -> VI Recorder16/2(Irec)
  Bus_13/1(Vabc) -> VI Recorder16/1(Vrec)
  connections:
  Bus Load 13/LConn1 -- CB3-2/LConn1 -- Bus_13/RConn1
  CB3-2/RConn3 -- OutPhaseC/RConn1
  Bus Load 13/LConn2 -- CB3-2/LConn2 -- Bus_13/RConn2
  Bus_13/RConn3 -- CB3-2/LConn3 -- Bus Load 13/LConn3
  CB3-2/RConn1 -- OutPhaseA/RConn1
  CB3-2/RConn2 -- OutPhaseB/RConn1
  InPhaseB/RConn1 -- Bus_13/LConn2
  Bus_13/LConn1 -- InPhaseA/RConn1
  InPhaseC/RConn1 -- Bus_13/LConn3

== system IEEE33_TR_TEMPORAL_RECOGNIZABILITY_MASTER/Bus_14 ==
  Bus Load 14 : Subsystem
      settings: AttributesFormatString=\n  OpenFcn=elec.conv.unmask(gcb);
  Bus_14 : Subsystem
      settings: OpenFcn=elec.conv.unmask(gcb);
  CB3-2 : Subsystem
      settings: OpenFcn=elec.conv.unmask(gcb);
  VI Recorder17 : Subsystem
  InPhaseA : PMIOPort  Side=Left
  InPhaseB : PMIOPort  Port=2  Side=Left
  InPhaseC : PMIOPort  Port=3  Side=Left
  OutPhaseA : PMIOPort  Port=4  Side=Right
  OutPhaseB : PMIOPort  Port=5  Side=Right
  OutPhaseC : PMIOPort  Port=6  Side=Right
  wires:
  [CB14to15] -> CB3-2/1(com)
  Bus_14/1(Vabc) -> VI Recorder17/1(Vrec)
  Bus_14/2(Iabc) -> VI Recorder17/2(Irec)
  connections:
  Bus_14/RConn1 -- CB3-2/LConn1 -- Bus Load 14/LConn1
  CB3-2/RConn3 -- OutPhaseC/RConn1
  Bus Load 14/LConn2 -- CB3-2/LConn2 -- Bus_14/RConn2
  Bus_14/RConn3 -- CB3-2/LConn3 -- Bus Load 14/LConn3
  CB3-2/RConn1 -- OutPhaseA/RConn1
  CB3-2/RConn2 -- OutPhaseB/RConn1
  InPhaseB/RConn1 -- Bus_14/LConn2
  InPhaseA/RConn1 -- Bus_14/LConn1
  InPhaseC/RConn1 -- Bus_14/LConn3

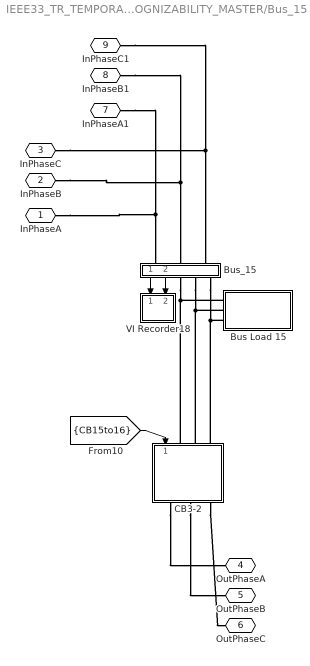
== system IEEE33_TR_TEMPORAL_RECOGNIZABILITY_MASTER/Bus_15 ==
  Bus Load 15 : Subsystem
      settings: AttributesFormatString=\n  OpenFcn=elec.conv.unmask(gcb);
  Bus_15 : Subsystem
      settings: OpenFcn=elec.conv.unmask(gcb);
  CB3-2 : Subsystem
      settings: OpenFcn=elec.conv.unmask(gcb);
  VI Recorder18 : Subsystem
  InPhaseA : PMIOPort  Side=Left
  InPhaseB : PMIOPort  Port=2  Side=Left
  InPhaseC : PMIOPort  Port=3  Side=Left
  OutPhaseA : PMIOPort  Port=4  Side=Right
  OutPhaseB : PMIOPort  Port=5  Side=Right
  OutPhaseC : PMIOPort  Port=6  Side=Right
  InPhaseA1 : PMIOPort  Port=7  Side=Left
  InPhaseB1 : PMIOPort  Port=8  Side=Left
  InPhaseC1 : PMIOPort  Port=9  Side=Left
  wires:
  [CB15to16] -> CB3-2/1(com)
  Bus_15/1(Vabc) -> VI Recorder18/1(Vrec)
  Bus_15/2(Iabc) -> VI Recorder18/2(Irec)
  connections:
  Bus Load 15/LConn1 -- CB3-2/LConn1 -- Bus_15/RConn1
  CB3-2/RConn3 -- OutPhaseC/RConn1
  Bus Load 15/LConn2 -- CB3-2/LConn2 -- Bus_15/RConn2
  Bus Load 15/LConn3 -- CB3-2/LConn3 -- Bus_15/RConn3
  CB3-2/RConn1 -- OutPhaseA/RConn1
  CB3-2/RConn2 -- OutPhaseB/RConn1
  InPhaseA1/RConn1 -- InPhaseA/RConn1 -- Bus_15/LConn1
  InPhaseB1/RConn1 -- InPhaseB/RConn1 -- Bus_15/LConn2
  InPhaseC1/RConn1 -- InPhaseC/RConn1 -- Bus_15/LConn3

== system IEEE33_TR_TEMPORAL_RECOGNIZABILITY_MASTER/Bus_16 ==
  Bus Load 16 : Subsystem
      settings: AttributesFormatString=\n  OpenFcn=elec.conv.unmask(gcb);
  Bus_16 : Subsystem
      settings: OpenFcn=elec.conv.unmask(gcb);
  CB3-2 : Subsystem
      settings: OpenFcn=elec.conv.unmask(gcb);
  VI Recorder19 : Subsystem
  InPhaseA : PMIOPort  Side=Left
  InPhaseB : PMIOPort  Port=2  Side=Left
  InPhaseC : PMIOPort  Port=3  Side=Left
  OutPhaseA : PMIOPort  Port=4  Side=Right
  OutPhaseB : PMIOPort  Port=5  Side=Right
  OutPhaseC : PMIOPort  Port=6  Side=Right
  wires:
  [CB16to17] -> CB3-2/1(com)
  Bus_16/1(Vabc) -> VI Recorder19/1(Vrec)
  Bus_16/2(Iabc) -> VI Recorder19/2(Irec)
  connections:
  Bus_16/RConn1 -- CB3-2/LConn1 -- Bus Load 16/LConn1
  CB3-2/RConn3 -- OutPhaseC/RConn1
  Bus Load 16/LConn2 -- CB3-2/LConn2 -- Bus_16/RConn2
  Bus Load 16/LConn3 -- CB3-2/LConn3 -- Bus_16/RConn3
  CB3-2/RConn1 -- OutPhaseA/RConn1
  CB3-2/RConn2 -- OutPhaseB/RConn1
  InPhaseC/RConn1 -- Bus_16/LConn3
  InPhaseB/RConn1 -- Bus_16/LConn2
  InPhaseA/RConn1 -- Bus_16/LConn1

== system IEEE33_TR_TEMPORAL_RECOGNIZABILITY_MASTER/Bus_17 ==
  Bus Load 17 : Subsystem
      settings: AttributesFormatString=\n  OpenFcn=elec.conv.unmask(gcb);
  Bus_17 : Subsystem
      settings: OpenFcn=elec.conv.unmask(gcb);
  CB3-2 : Subsystem
      settings: OpenFcn=elec.conv.unmask(gcb);
  VI Recorder20 : Subsystem
  InPhaseA : PMIOPort  Side=Left
  InPhaseB : PMIOPort  Port=2  Side=Left
  InPhaseC : PMIOPort  Port=3  Side=Left
  OutPhaseA : PMIOPort  Port=4  Side=Right
  OutPhaseB : PMIOPort  Port=5  Side=Right
  OutPhaseC : PMIOPort  Port=6  Side=Right
  wires:
  [CB17to18] -> CB3-2/1(com)
  Bus_17/2(Iabc) -> VI Recorder20/2(Irec)
  Bus_17/1(Vabc) -> VI Recorder20/1(Vrec)
  connections:
  Bus_17/RConn1 -- CB3-2/LConn1 -- Bus Load 17/LConn1
  CB3-2/RConn3 -- OutPhaseC/RConn1
  Bus Load 17/LConn2 -- CB3-2/LConn2 -- Bus_17/RConn2
  Bus_17/RConn3 -- CB3-2/LConn3 -- Bus Load 17/LConn3
  CB3-2/RConn1 -- OutPhaseA/RConn1
  CB3-2/RConn2 -- OutPhaseB/RConn1
  InPhaseA/RConn1 -- Bus_17/LConn1
  InPhaseB/RConn1 -- Bus_17/LConn2
  InPhaseC/RConn1 -- Bus_17/LConn3

== system IEEE33_TR_TEMPORAL_RECOGNIZABILITY_MASTER/Bus_18 ==
  Bus Load 18 : Subsystem
      settings: AttributesFormatString=\n  OpenFcn=elec.conv.unmask(gcb);
  Bus_18 : Subsystem
      settings: OpenFcn=elec.conv.unmask(gcb);
  CB3-2 : Subsystem
      settings: OpenFcn=elec.conv.unmask(gcb);
  VI Recorder21 : Subsystem
  InPhaseA : PMIOPort  Side=Left
  InPhaseB : PMIOPort  Port=2  Side=Left
  InPhaseC : PMIOPort  Port=3  Side=Left
  OutPhaseA : PMIOPort  Port=4  Side=Right
  OutPhaseB : PMIOPort  Port=5  Side=Right
  OutPhaseC : PMIOPort  Port=6  Side=Right
  wires:
  [CB18to33] -> CB3-2/1(com)
  Bus_18/1(Vabc) -> VI Recorder21/1(Vrec)
  Bus_18/2(Iabc) -> VI Recorder21/2(Irec)
  connections:
  Bus_18/RConn1 -- CB3-2/LConn1 -- Bus Load 18/LConn1
  CB3-2/RConn3 -- OutPhaseC/RConn1
  Bus Load 18/LConn2 -- CB3-2/LConn2 -- Bus_18/RConn2
  Bus Load 18/LConn3 -- CB3-2/LConn3 -- Bus_18/RConn3
  CB3-2/RConn1 -- OutPhaseA/RConn1
  CB3-2/RConn2 -- OutPhaseB/RConn1
  InPhaseA/RConn1 -- Bus_18/LConn1
  InPhaseB/RConn1 -- Bus_18/LConn2
  InPhaseC/RConn1 -- Bus_18/LConn3

== system IEEE33_TR_TEMPORAL_RECOGNIZABILITY_MASTER/Bus_19 ==
  Bus Load 19 : Subsystem
      settings: AttributesFormatString=\n  OpenFcn=elec.conv.unmask(gcb);
  Bus_19 : Subsystem
      settings: OpenFcn=elec.conv.unmask(gcb);
  CB3-2 : Subsystem
      settings: OpenFcn=elec.conv.unmask(gcb);
  VI Recorder : Subsystem
  InPhaseA : PMIOPort  Side=Left
  InPhaseB : PMIOPort  Port=2  Side=Left
  InPhaseC : PMIOPort  Port=3  Side=Left
  OutPhaseA : PMIOPort  Port=4  Side=Right
  OutPhaseB : PMIOPort  Port=5  Side=Right
  OutPhaseC : PMIOPort  Port=6  Side=Right
  wires:
  [CB19to20] -> CB3-2/1(com)
  Bus_19/2(Iabc) -> VI Recorder/2(Irec)
  Bus_19/1(Vabc) -> VI Recorder/1(Vrec)
  connections:
  Bus_19/RConn1 -- CB3-2/LConn1 -- Bus Load 19/LConn1
  CB3-2/RConn3 -- OutPhaseC/RConn1
  Bus Load 19/LConn2 -- CB3-2/LConn2 -- Bus_19/RConn2
  Bus_19/RConn3 -- CB3-2/LConn3 -- Bus Load 19/LConn3
  CB3-2/RConn1 -- OutPhaseA/RConn1
  CB3-2/RConn2 -- OutPhaseB/RConn1
  Bus_19/LConn1 -- InPhaseA/RConn1
  InPhaseB/RConn1 -- Bus_19/LConn2
  InPhaseC/RConn1 -- Bus_19/LConn3

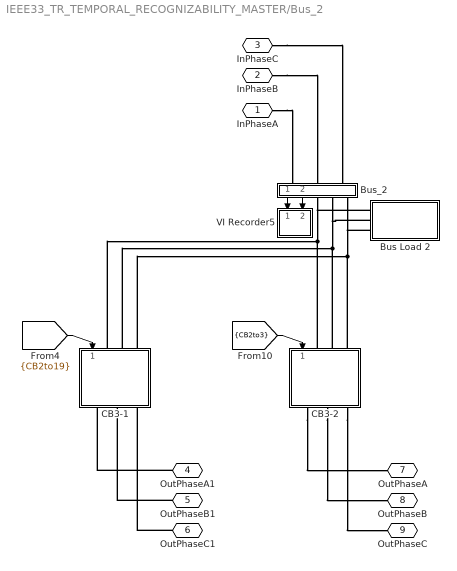
== system IEEE33_TR_TEMPORAL_RECOGNIZABILITY_MASTER/Bus_2 ==
  Bus Load 2 : Subsystem
      settings: AttributesFormatString=\n  OpenFcn=elec.conv.unmask(gcb);
  Bus_2 : Subsystem
      settings: OpenFcn=elec.conv.unmask(gcb);
  CB3-1 : Subsystem
      settings: OpenFcn=elec.conv.unmask(gcb);
  CB3-2 : Subsystem
      settings: OpenFcn=elec.conv.unmask(gcb);
  VI Recorder5 : Subsystem
  InPhaseA : PMIOPort  Side=Left
  InPhaseB : PMIOPort  Port=2  Side=Left
  InPhaseC : PMIOPort  Port=3  Side=Left
  OutPhaseA1 : PMIOPort  Port=4  Side=Right
  OutPhaseB1 : PMIOPort  Port=5  Side=Right
  OutPhaseC1 : PMIOPort  Port=6  Side=Right
  OutPhaseA : PMIOPort  Port=7  Side=Right
  OutPhaseB : PMIOPort  Port=8  Side=Right
  OutPhaseC : PMIOPort  Port=9  Side=Right
  wires:
  [CB2to3] -> CB3-2/1(com)
  Bus_2/2(Iabc) -> VI Recorder5/2(Irec)
  Bus_2/1(Vabc) -> VI Recorder5/1(Vrec)
  [CB2to19] -> CB3-1/1(com)
  connections:
  CB3-1/LConn1 -- CB3-2/LConn1 -- Bus Load 2/LConn1 -- Bus_2/RConn1
  CB3-1/LConn2 -- Bus Load 2/LConn2 -- Bus_2/RConn2 -- CB3-2/LConn2
  CB3-1/LConn3 -- Bus Load 2/LConn3 -- Bus_2/RConn3 -- CB3-2/LConn3
  InPhaseC/RConn1 -- Bus_2/LConn3
  InPhaseB/RConn1 -- Bus_2/LConn2
  InPhaseA/RConn1 -- Bus_2/LConn1
  OutPhaseA1/RConn1 -- CB3-1/RConn1
  OutPhaseC1/RConn1 -- CB3-1/RConn3
  OutPhaseB1/RConn1 -- CB3-1/RConn2
  CB3-2/RConn1 -- OutPhaseA/RConn1
  CB3-2/RConn2 -- OutPhaseB/RConn1
  CB3-2/RConn3 -- OutPhaseC/RConn1

== system IEEE33_TR_TEMPORAL_RECOGNIZABILITY_MASTER/Bus_20 ==
  Bus Load 20 : Subsystem
      settings: AttributesFormatString=\n  OpenFcn=elec.conv.unmask(gcb);
  Bus_20 : Subsystem
      settings: OpenFcn=elec.conv.unmask(gcb);
  CB3-2 : Subsystem
      settings: OpenFcn=elec.conv.unmask(gcb);
  VI Recorder1 : Subsystem
  InPhaseA : PMIOPort  Side=Left
  InPhaseB : PMIOPort  Port=2  Side=Left
  InPhaseC : PMIOPort  Port=3  Side=Left
  OutPhaseA : PMIOPort  Port=4  Side=Right
  OutPhaseB : PMIOPort  Port=5  Side=Right
  OutPhaseC : PMIOPort  Port=6  Side=Right
  wires:
  [CB20to21] -> CB3-2/1(com)
  Bus_20/1(Vabc) -> VI Recorder1/1(Vrec)
  Bus_20/2(Iabc) -> VI Recorder1/2(Irec)
  connections:
  Bus_20/RConn1 -- CB3-2/LConn1 -- Bus Load 20/LConn1
  CB3-2/RConn3 -- OutPhaseC/RConn1
  Bus Load 20/LConn2 -- CB3-2/LConn2 -- Bus_20/RConn2
  Bus_20/RConn3 -- CB3-2/LConn3 -- Bus Load 20/LConn3
  CB3-2/RConn1 -- OutPhaseA/RConn1
  CB3-2/RConn2 -- OutPhaseB/RConn1
  InPhaseA/RConn1 -- Bus_20/LConn1
  InPhaseB/RConn1 -- Bus_20/LConn2
  InPhaseC/RConn1 -- Bus_20/LConn3

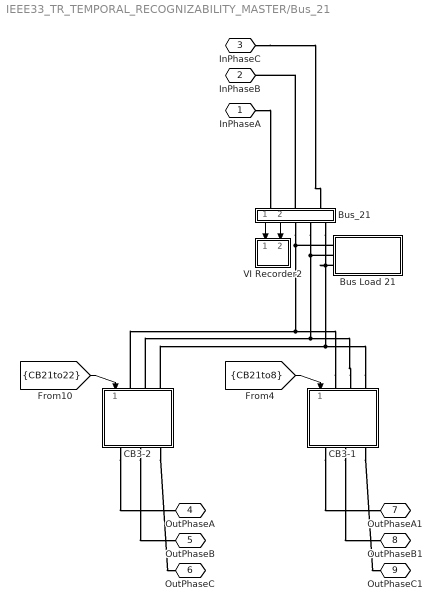
== system IEEE33_TR_TEMPORAL_RECOGNIZABILITY_MASTER/Bus_21 ==
  Bus Load 21 : Subsystem
      settings: AttributesFormatString=\n  OpenFcn=elec.conv.unmask(gcb);
  Bus_21 : Subsystem
      settings: OpenFcn=elec.conv.unmask(gcb);
  CB3-1 : Subsystem
      settings: OpenFcn=elec.conv.unmask(gcb);
  CB3-2 : Subsystem
      settings: OpenFcn=elec.conv.unmask(gcb);
  VI Recorder2 : Subsystem
  InPhaseA : PMIOPort  Side=Left
  InPhaseB : PMIOPort  Port=2  Side=Left
  InPhaseC : PMIOPort  Port=3  Side=Left
  OutPhaseA : PMIOPort  Port=4  Side=Right
  OutPhaseB : PMIOPort  Port=5  Side=Right
  OutPhaseC : PMIOPort  Port=6  Side=Right
  OutPhaseA1 : PMIOPort  Port=7  Side=Right
  OutPhaseB1 : PMIOPort  Port=8  Side=Right
  OutPhaseC1 : PMIOPort  Port=9  Side=Right
  wires:
  [CB21to22] -> CB3-2/1(com)
  Bus_21/2(Iabc) -> VI Recorder2/2(Irec)
  Bus_21/1(Vabc) -> VI Recorder2/1(Vrec)
  [CB21to8] -> CB3-1/1(com)
  connections:
  CB3-1/LConn1 -- Bus Load 21/LConn1 -- Bus_21/RConn1 -- CB3-2/LConn1
  CB3-2/RConn3 -- OutPhaseC/RConn1
  CB3-1/LConn2 -- Bus Load 21/LConn2 -- Bus_21/RConn2 -- CB3-2/LConn2
  CB3-1/LConn3 -- Bus_21/RConn3 -- Bus Load 21/LConn3 -- CB3-2/LConn3
  CB3-2/RConn1 -- OutPhaseA/RConn1
  CB3-2/RConn2 -- OutPhaseB/RConn1
  InPhaseA/RConn1 -- Bus_21/LConn1
  Bus_21/LConn2 -- InPhaseB/RConn1
  InPhaseC/RConn1 -- Bus_21/LConn3
  CB3-1/RConn3 -- OutPhaseC1/RConn1
  CB3-1/RConn1 -- OutPhaseA1/RConn1
  CB3-1/RConn2 -- OutPhaseB1/RConn1
